simulink model "Controller"  (R2026b)
settings: Solver=VariableStepAuto
undefined symbols (not defined in the file): DiscIntNeverNeededParam, input_filter
libraries: slpidlib x2
settings Model: Creator=Dani  LastModifiedBy=Dani

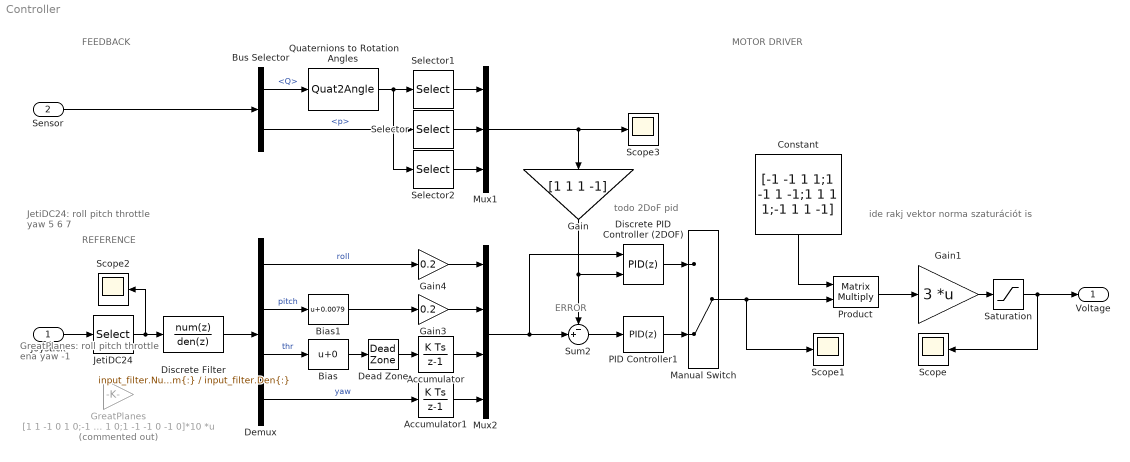
== system Controller ==
  note: todo 2DoF pid
  note: MOTOR DRIVER
  note: ERROR
  note: REFERENCE
  note: FEEDBACK
  note: ide rakj vektor norma szaturációt is
  note: JetiDC24:
      |
      | roll
      | pitch
      | throttle
      | yaw
      | 5
      | 6
      | 7
  note: GreatPlanes:
      |
      | roll
      | pitch
      | throttle
      | ena
      | yaw
      | -1
  Joystick : Inport
  Sensor : Inport  Port=2
  Accumulator : DiscreteIntegrator  gainval=0.5  InitialCondition=0.350  SampleTime=-1  LimitOutput=on  UpperSaturationLimit=1.85  LowerSaturationLimit=0.0251535  ICPrevOutput=DiscIntNeverNeededParam  ICPrevScaledInput=DiscIntNeverNeededParam
  Accumulator1 : DiscreteIntegrator  gainval=0.2  InitialCondition=0.350  SampleTime=-1  UpperSaturationLimit=0.2  ICPrevOutput=DiscIntNeverNeededParam  ICPrevScaledInput=DiscIntNeverNeededParam
  Bias : Bias  SaturateOnIntegerOverflow=off
  Bias1 : Bias  Bias=0.0079  SaturateOnIntegerOverflow=off
  Bus Selector : BusSelector  OutputSignals=States.Q,States.p
  Constant : Constant  Value=[-1 -1 1 1;1 -1 1 -1;1 1 1 1;-1 1 1 -1]
  Dead Zone : DeadZone  LowerValue=-0.2  UpperValue=0.2  ZeroCross=off
  Demux : Demux
  Discrete Filter : DiscreteFilter  Numerator=input_filter.Num{:}  Denominator=input_filter.Den{:}
  Discrete PID Controller (2DOF) : slpidlib/PID Controller (2DOF)  Controller=PID  Form=Parallel  TimeDomain=Discrete-time  UseExternalTs=off  SampleTime=-1  IntegratorMethod=Forward Euler  FilterMethod=Forward Euler  ControllerParametersSource=internal  P=[0.1 0.5 3 1]  I=1  UseKiTs=off  D=0  UseExternalDerivativeSource=off  N=100  UseFilter=on  b=1  c=1  TunerSelectOption=Transfer Function Based (PID Tuner App)  InitialConditionSource=internal  InitialConditionForIntegrator=0  InitialConditionForFilter=0  DifferentiatorICPrevScaledInput=0  ExternalReset=none  TrackingMode=off  Kt=1  LimitOutput=off  SatLimitsSource=internal  UpperSaturationLimit=inf  LowerSaturationLimit=-inf  LinearizeAsGain=off  AntiWindupMode=none  Kb=1  LimitIntegrator=off  UpperIntegratorSaturationLimit=inf  LowerIntegratorSaturationLimit=-inf  POutMin=[]  POutMax=[]  IOutMin=[]  IOutMax=[]  DOutMin=[]  DOutMax=[]  NOutMin=[]  NOutMax=[]  bOutMin=[]  bOutMax=[]  cOutMin=[]  cOutMax=[]  SumOutMin=[]  SumOutMax=[]  SaturationOutMin=[]  SaturationOutMax=[]  PParamMin=[]  PParamMax=[]  IParamMin=[]  IParamMax=[]  DParamMin=[]  DParamMax=[]  NParamMin=[]  NParamMax=[]  bParamMin=[]  bParamMax=[]  cParamMin=[]  cParamMax=[]  KbParamMin=[]  KbParamMax=[]  KtParamMin=[]  KtParamMax=[]  KbOutMin=[]  KbOutMax=[]  KtOutMin=[]  KtOutMax=[]  IntegratorOutMin=[]  IntegratorOutMax=[]  FilterOutMin=[]  FilterOutMax=[]  SumI1OutMin=[]  SumI1OutMax=[]  SumI2OutMin=[]  SumI2OutMax=[]  SumI3OutMin=[]  SumI3OutMax=[]  SumI4OutMin=[]  SumI4OutMax=[]  SumDOutMin=[]  SumDOutMax=[]  Sum1OutMin=[]  Sum1OutMax=[]  Sum2OutMin=[]  Sum2OutMax=[]  Sum3OutMin=[]  Sum3OutMax=[]  DifferentiatorOutMin=[]  DifferentiatorOutMax=[]  FilterDiffOutCoefMin=[]  FilterDiffOutCoefMax=[]  ReciprocalOutMin=[]  ReciprocalOutMax=[]  SumDenOutMin=[]  SumDenOutMax=[]  SumNumOutMin=[]  SumNumOutMax=[]  DivideOutMin=[]  DivideOutMax=[]  UdiffTsProdOutMin=[]  UdiffTsProdOutMax=[]  NTsProdOutMin=[]  NTsProdOutMax=[]  UintegralTsProdOutMin=[]  UintegralTsProdOutMax=[]  UngainTsProdOutMin=[]  UngainTsProdOutMax=[]  ClampingZeroOutDataTypeStr=Inherit: Inherit via back propagation  ClampingZeroOutMin=[]  ClampingZeroOutMax=[]  FilterDenConstantOutDataTypeStr=Inherit: Inherit via back propagation  FilterDenConstantOutMin=[]  FilterDenConstantOutMax=[]  PCopyOutDataTypeStr=Inherit: Inherit via back propagation  PCopyOutMin=[]  PCopyOutMax=[]  NCopyOutDataTypeStr=Inherit: Inherit via back propagation  NCopyOutMin=[]  NCopyOutMax=[]  IntegratorContinuousStateAttributes=''  IntegratorStateMustResolveToSignalObject=off  IntegratorRTWStateStorageClass=Auto  FilterContinuousStateAttributes=''  FilterStateMustResolveToSignalObject=off  FilterRTWStateStorageClass=Auto  ParallelPVariant=InternalParameters  IdealPVariant=Disabled  IVariant=InternalParameters  DVariant=InternalParameters  bVariant=InternalParameters  cVariant=InternalParameters  IntegratorVariant=Discrete  SatVariant=Disabled  AWVariant=Passthrough  PCopyVariant=Disabled  TRVariant=Disabled  FdbkBlocksVariant=Forward  IdealPFdbkVariant=Disabled  SatFdbkVariant=Disabled  DerivativeFilterVariant=ForwardEulerFilter  NVariant=InternalParameters  NCopyVariant=Disabled  FilterICVariant=InternalICsFilter  IntegratorICVariant=InternalICs  ExternalResetVariant=Disabled  TRSumVariant=Passthrough  SumFdbkVariant=Disabled  SumVariant=Sum_PID  TsampFilterVariant=InternalTs  TsampNgainVariant=Passthrough  TsampIntegralVariant=Disabled_SignalSpec  ExternalSaturationOutDataTypeStr=Inherit: Same as second input  DerivativeSourceVariant=ErrorSignal  PreIntVariant=InternalPreInt
      settings: LibrarySourceBlock=simulink/Discrete/Discrete PID Controller (2DOF)
  Gain : Gain  Gain=[1 1 1 -1]
  Gain1 : Gain  Gain=3  Multiplication=Matrix(K*u)
  Gain3 : Gain  Gain=0.2
  Gain4 : Gain  Gain=0.2
  GreatPlanes : Gain  Commented=on  Gain=[1 1 -1 0 1 0;-1 1 -1 0 -1 0;-1 -1 -1 0 1 0;1 -1 -1 0 -1 0]*10  Multiplication=Matrix(K*u)
  JetiDC24 : Selector  IndexOptions=Index vector (dialog)  Indices=1:4  OutputSizes=1
  Manual Switch : ManualSwitch  CurrentSetting=0
  Mux1 : Mux  Inputs=3
  Mux2 : Mux
  PID Controller1 : slpidlib/PID Controller  Controller=PID  Form=Parallel  TimeDomain=Discrete-time  UseExternalTs=off  SampleTime=-1  IntegratorMethod=Forward Euler  FilterMethod=Forward Euler  ControllerParametersSource=internal  P=[0.1 0.5 3 0.3]  I=[0.1 0.1 0.1 0]  UseKiTs=off  D=[0.2 0.2 1 0.2]  UseExternalDerivativeSource=off  N=100  UseFilter=on  TunerSelectOption=Transfer Function Based (PID Tuner App)  InitialConditionSource=internal  InitialConditionForIntegrator=[0 0 1.33 0]  InitialConditionForFilter=0  DifferentiatorICPrevScaledInput=0  ExternalReset=none  TrackingMode=off  Kt=1  LimitOutput=off  SatLimitsSource=internal  UpperSaturationLimit=inf  LowerSaturationLimit=-inf  LinearizeAsGain=on  AntiWindupMode=none  Kb=1  LimitIntegrator=off  UpperIntegratorSaturationLimit=100  LowerIntegratorSaturationLimit=-100  POutMin=[]  POutMax=[]  IOutMin=[]  IOutMax=[]  DOutMin=[]  DOutMax=[]  NOutMin=[]  NOutMax=[]  SumOutMin=[]  SumOutMax=[]  SaturationOutMin=[]  SaturationOutMax=[]  PParamMin=[]  PParamMax=[]  IParamMin=[]  IParamMax=[]  DParamMin=[]  DParamMax=[]  NParamMin=[]  NParamMax=[]  KbParamMin=[]  KbParamMax=[]  KtParamMin=[]  KtParamMax=[]  KbOutMin=[]  KbOutMax=[]  KtOutMin=[]  KtOutMax=[]  IntegratorOutMin=[]  IntegratorOutMax=[]  FilterOutMin=[]  FilterOutMax=[]  SumI1OutMin=[]  SumI1OutMax=[]  SumI2OutMin=[]  SumI2OutMax=[]  SumI3OutMin=[]  SumI3OutMax=[]  SumI4OutMin=[]  SumI4OutMax=[]  SumDOutMin=[]  SumDOutMax=[]  DifferentiatorOutMin=[]  DifferentiatorOutMax=[]  FilterDiffOutCoefMin=[]  FilterDiffOutCoefMax=[]  ReciprocalOutMin=[]  ReciprocalOutMax=[]  SumDenOutMin=[]  SumDenOutMax=[]  SumNumOutMin=[]  SumNumOutMax=[]  DivideOutMin=[]  DivideOutMax=[]  UdiffTsProdOutMin=[]  UdiffTsProdOutMax=[]  NTsProdOutMin=[]  NTsProdOutMax=[]  UintegralTsProdOutMin=[]  UintegralTsProdOutMax=[]  UngainTsProdOutMin=[]  UngainTsProdOutMax=[]  ClampingZeroOutDataTypeStr=Inherit: Inherit via back propagation  ClampingZeroOutMin=[]  ClampingZeroOutMax=[]  FilterDenConstantOutDataTypeStr=Inherit: Inherit via back propagation  FilterDenConstantOutMin=[]  FilterDenConstantOutMax=[]  PCopyOutDataTypeStr=Inherit: Inherit via back propagation  PCopyOutMin=[]  PCopyOutMax=[]  NCopyOutDataTypeStr=Inherit: Inherit via back propagation  NCopyOutMin=[]  NCopyOutMax=[]  IntegratorContinuousStateAttributes=''  IntegratorStateMustResolveToSignalObject=off  IntegratorRTWStateStorageClass=Auto  FilterContinuousStateAttributes=''  FilterStateMustResolveToSignalObject=off  FilterRTWStateStorageClass=Auto  ParallelPVariant=InternalParameters  IdealPVariant=Disabled  IVariant=InternalParameters  DVariant=InternalParameters  IntegratorVariant=Discrete  SatVariant=Disabled  AWVariant=Passthrough  PCopyVariant=Disabled  TRVariant=Disabled  FdbkBlocksVariant=Forward  IdealPFdbkVariant=Disabled  SatFdbkVariant=Disabled  DerivativeFilterVariant=ForwardEulerFilter  NVariant=InternalParameters  NCopyVariant=Disabled  FilterICVariant=InternalICsFilter  IntegratorICVariant=InternalICs  ExternalResetVariant=Disabled  TRSumVariant=Passthrough  SumFdbkVariant=Disabled  SumVariant=Sum_PID  TsampFilterVariant=InternalTs  TsampNgainVariant=Passthrough  TsampIntegralVariant=Disabled_SignalSpec  ExternalSaturationOutDataTypeStr=Inherit: Same as second input  DerivativeSourceVariant=ErrorSignal  PreIntVariant=InternalPreInt
  Product : Product  Multiplication=Matrix(*)
  Quaternions to Rotation Angles : Quat2Angle  rotationOrder=XYZ
      settings: AttributesFormatString=Rotation Order: %<rotationOrder>
  Saturation : Saturate  UpperLimit=16  LowerLimit=-16*0
  Scope{,1..3} (4 alike) : Scope
      Scope settings: ActiveDisplayYMinimum=3.9267341625213881  ActiveDisplayYMaximum=3.9285492485275362  DataLoggingVariableName=ScopeData3
      Scope1 settings: ActiveDisplayYMinimum=-0.084590678413535514  ActiveDisplayYMaximum=0.11475618543817268  DataLoggingVariableName=ScopeData2
      Scope2 settings: ActiveDisplayYMinimum=-0.9892461935435215  ActiveDisplayYMaximum=0.94451148958284814  DataLoggingVariableName=ScopeData4
      Scope3 settings: ActiveDisplayYMinimum=-4.0973693882839077  ActiveDisplayYMaximum=4.5604751007887527  DataLoggingVariableName=ScopeData6
  Selector : Selector  InputPortWidth=3  IndexOptions=Index vector (dialog)  Indices=3  OutputSizes=1
  Selector1 : Selector  InputPortWidth=3  IndexOptions=Index vector (dialog)  Indices=Euler_selector  OutputSizes=1
  Selector2 : Selector  InputPortWidth=3  IndexOptions=Index vector (dialog)  Indices=Euler_selectorZ  OutputSizes=1
  Sum2 : Sum  Inputs=-+|
  Voltage : Outport
  wires:
  Joystick/1 -> JetiDC24/1
  Demux/1 -> Gain4/1  "roll"
  Demux/2 -> Bias1/1  "pitch"
  Demux/3 -> Bias/1  "thr"
  Demux/4 -> Accumulator1/1  "yaw"
  JetiDC24/1 -> Discrete Filter/1, Scope2/1
  Product/1 -> Gain1/1
  Constant/1 -> Product/1
  Manual Switch/1 -> Product/2, Scope1/1
  Gain1/1 -> Saturation/1
  Saturation/1 -> Voltage/1, Scope/1
  Bias1/1 -> Gain3/1
  Sensor/1 -> Bus Selector/1
  Accumulator/1 -> Mux2/3
  Sum2/1 -> PID Controller1/1
  Quaternions to Rotation Angles/1 -> Selector2/1, Selector1/1
  Mux1/1 -> Gain/1, Scope3/1
  Gain4/1 -> Mux2/1
  Gain3/1 -> Mux2/2
  Selector/1 -> Mux1/2
  Bias/1 -> Dead Zone/1
  Mux2/1 -> Discrete PID Controller (2DOF)/1, Sum2/2
  Dead Zone/1 -> Accumulator/1
  Selector1/1 -> Mux1/1
  Discrete Filter/1 -> Demux/1
  Accumulator1/1 -> Mux2/4
  Selector2/1 -> Mux1/3
  PID Controller1/1 -> Manual Switch/2
  Discrete PID Controller (2DOF)/1 -> Manual Switch/1
  Bus Selector/2 -> Selector/1  "<p>"
  Bus Selector/1 -> Quaternions to Rotation Angles/1  "<Q>"
  Gain/1 -> Sum2/1, Discrete PID Controller (2DOF)/2
